simulink model "untitled"  (R2023a)
settings: Solver=VariableStepAuto  StartTime=0.0  StopTime=10.0  RelTol=1e-3
settings Model: Creator=natew  LastModifiedBy=natew

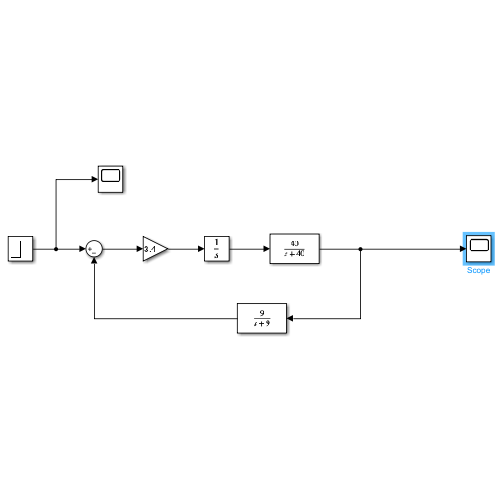
[thumbnail: Simulink's stored preview of the top-level diagram]
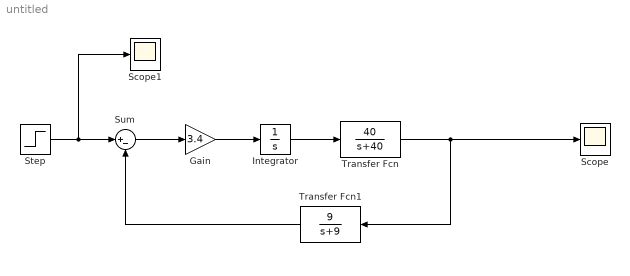
== system untitled ==
  Gain : Gain  Gain=3.4
  Integrator : Integrator
  Scope : Scope
  Scope1 : Scope
  Step : Step  Time=.0001  SampleTime=0
  Sum : Sum  Inputs=|+-
  Transfer Fcn : TransferFcn  Numerator=[40]  Denominator=[1 40]
  Transfer Fcn1 : TransferFcn  Numerator=[9]  Denominator=[1 9]
  wires:
  Transfer Fcn1/1 -> Sum/2
  Integrator/1 -> Transfer Fcn/1
  Transfer Fcn/1 -> Transfer Fcn1/1, Scope/1
  Step/1 -> Scope1/1, Sum/1
  Gain/1 -> Integrator/1
  Sum/1 -> Gain/1
